simulink model "Transmission_Line_132kV_Phase1"  (R2024b)
settings: Solver=FixedStepDiscrete  StartTime=0.0  StopTime=0.40000000000000002  FixedStep=2e-05  RelTol=1e-3
libraries: spsThreePhasePISectionLineLib x2, spsThreePhaseVIMeasurementLib x2, spsThreePhaseFaultLib x1, spsThreePhaseParallelRLCLoadLib x1, spsThreePhaseSourceLib x1, sps_lib x1
settings Model: Creator=Raju  LastModifiedBy=Raju

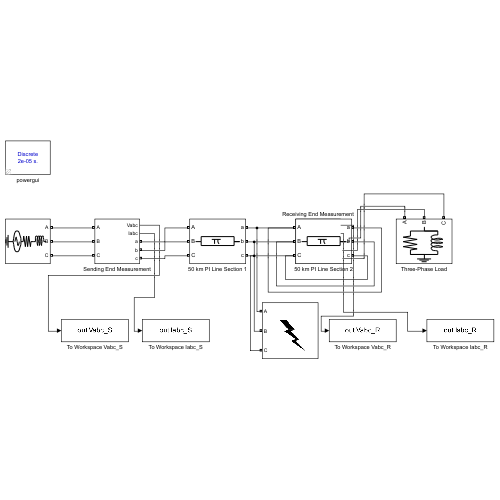
[thumbnail: Simulink's stored preview of the top-level diagram]
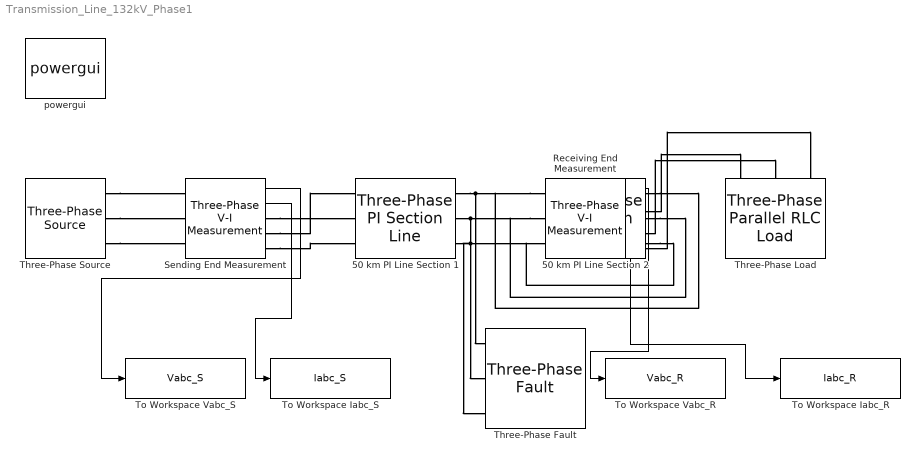
== system Transmission_Line_132kV_Phase1 ==
  50 km PI Line Section 1 : spsThreePhasePISectionLineLib/Three-Phase PI Section Line  LConnTagsString=a|b|c  RConnTagsString=A|B|C  Length=50  Frequency=50  Resistances=[0.03 0.3]  Inductances=[0.001 0.003]  Capacitances=[1.2e-08 6e-09]
  50 km PI Line Section 2 : spsThreePhasePISectionLineLib/Three-Phase PI Section Line  LConnTagsString=a|b|c  RConnTagsString=A|B|C  Length=50  Frequency=50  Resistances=[0.03 0.3]  Inductances=[0.001 0.003]  Capacitances=[1.2e-08 6e-09]
  Receiving End Measurement : spsThreePhaseVIMeasurementLib/Three-Phase V-I Measurement  VoltageMeasurement=phase-to-ground  SetLabelV=off  LabelV=Vabc  Vpu=off  VpuLL=off  CurrentMeasurement=yes  SetLabelI=off  LabelI=Iabc  Ipu=off  Pbase=100e6  Vbase=500e3  OutputType=Complex  PhasorSimulation=off  PSBequivalent=0
  Sending End Measurement : spsThreePhaseVIMeasurementLib/Three-Phase V-I Measurement  VoltageMeasurement=phase-to-ground  SetLabelV=off  LabelV=Vabc  Vpu=off  VpuLL=off  CurrentMeasurement=yes  SetLabelI=off  LabelI=Iabc  Ipu=off  Pbase=100e6  Vbase=500e3  OutputType=Complex  PhasorSimulation=off  PSBequivalent=0
  Three-Phase Fault : spsThreePhaseFaultLib/Three-Phase Fault  InitialStates=0  FaultA=on  FaultB=on  FaultC=on  GroundFault=on  SwitchTimes=[0.10 0.20]  External=off  SwitchStatus=NaN  FaultResistance=0.001  GroundResistance=0.001  SnubberResistance=1e6  SnubberCapacitance=inf  Measurements=None
  Three-Phase Load : spsThreePhaseParallelRLCLoadLib/Three-Phase Parallel RLC Load  LConnTagsString=A|B|C  Configuration=Y (grounded)  NominalVoltage=132000  Vabc=[1e3 1e3 1e3]  Vabcp=[1e3 1e3 1e3]  NominalFrequency=50  UnbalancedPower=off  ActivePower=50000000  InductivePower=16434205.258943161  CapacitivePower=0  Pabc=[10e3 9e3 11e3]  QLabc=[100 90 110]  QCabc=[100 90 110]  Pabcp=[10e3 9e3 11e3]  QLabcp=[100 90 110]  QCabcp=[100 90 110]  Measurements=None  LoadType=constant PQ
  Three-Phase Source : spsThreePhaseSourceLib/Three-Phase Source  InternalConnection=Yg  VoltagePhases=off  Voltage=132000  PhaseAngle=0  Voltage_phases=[25e3 25e3 25e3]/sqrt(3)  PhaseAngles_phases=[0 -120 +120]  Frequency=50  NonIdealSource=on  SpecifyImpedance=on  Resistance=0.8929  Inductance=16.58e-3  ShortCircuitLevel=1000000000  BaseVoltage=132000  XRratio=10  BusType=swing  Pref=10e3  Qref=0  Prefabc=[10e3, 10e3, 10e3]  Qrefabc=[0, 0, 0]  Qmin=-inf  Qmax=inf
  To Workspace Iabc_R : ToWorkspace  VariableName=Iabc_R  SaveFormat=Timeseries  SampleTime=-1
  To Workspace Iabc_S : ToWorkspace  VariableName=Iabc_S  SaveFormat=Timeseries  SampleTime=-1
  To Workspace Vabc_R : ToWorkspace  VariableName=Vabc_R  SaveFormat=Timeseries  SampleTime=-1
  To Workspace Vabc_S : ToWorkspace  VariableName=Vabc_S  SaveFormat=Timeseries  SampleTime=-1
  powergui : sps_lib/powergui  Priority=1  SimulationMode=Discrete  SampleTime=2.0000000000000002e-05  frequency=60  Iterations=50  frequencyindice=50  Pbase=100e6  ErrMax=1e-4  UnitsV=kV  UnitsW=MW  buscounter=0  FunctionMessages=off  echomessages=off  EnableUseOfTLC=off  CurrentSourceSwitches=off  DisableSnubberDevices=off  DisableRonSwitches=off  DisableVfSwitches=off  DisplayEquations=off  AutomaticDiscreteSolvers=off  SolverType=Tustin/Backward Euler (TBE)  Interpol=off  ExternalGateDelay=off  methode=off  Ts=100  x0status=blocks  SPID=on  SwTol=0  HookPort=off  NonlinearTolerance=1e-4  nMaxIteration=100  ContinueOnMaxIteration=off  RestoreLinks=warning  ResistiveCurrentMeasurement=off  Frange=[0:2:500]  Ylog=off  Xlog=on  ShowGrid=off  save=off  variable=ZData  structure=0  ZoomFFT=off  StartTime=0.0  cycles=1  DisplayStyle=1  fundamental=60  FreqAxis=off  MaxFrequency=1000  frequencyindicesteady=1  RmsSteady=1  display=off
  wires:
  Sending End Measurement/1 -> To Workspace Vabc_S/1
  Sending End Measurement/2 -> To Workspace Iabc_S/1
  Receiving End Measurement/1 -> To Workspace Vabc_R/1
  Receiving End Measurement/2 -> To Workspace Iabc_R/1
  connections:
  Three-Phase Source/RConn1 -- Sending End Measurement/LConn1
  Sending End Measurement/RConn1 -- 50 km PI Line Section 1/LConn1
  50 km PI Line Section 2/RConn1 -- Receiving End Measurement/LConn1
  Receiving End Measurement/RConn1 -- Three-Phase Load/LConn1
  Three-Phase Source/RConn2 -- Sending End Measurement/LConn2
  Sending End Measurement/RConn2 -- 50 km PI Line Section 1/LConn2
  50 km PI Line Section 2/RConn2 -- Receiving End Measurement/LConn2
  Receiving End Measurement/RConn2 -- Three-Phase Load/LConn2
  Three-Phase Source/RConn3 -- Sending End Measurement/LConn3
  Sending End Measurement/RConn3 -- 50 km PI Line Section 1/LConn3
  50 km PI Line Section 2/RConn3 -- Receiving End Measurement/LConn3
  Receiving End Measurement/RConn3 -- Three-Phase Load/LConn3
  50 km PI Line Section 2/LConn1 -- 50 km PI Line Section 1/RConn1 -- Three-Phase Fault/LConn1
  50 km PI Line Section 2/LConn2 -- 50 km PI Line Section 1/RConn2 -- Three-Phase Fault/LConn2
  50 km PI Line Section 1/RConn3 -- 50 km PI Line Section 2/LConn3 -- Three-Phase Fault/LConn3
